simulink model "HPP"  (R2026a)
settings: Solver=ode1  StopTime=p.sim.Tstop  FixedStep=HPP_Tnet
model workspace (MAT data in the model file):
  HPP_Tnet = 0.001
  HPP_Ts = 0.001
  HPP_delays = 1
  HPP_f0 = 50
  HPP_network = 1
  HPP_simscape = 1
  buildInfo.N_wt = 2
  buildInfo.N_pv = 2
  buildInfo.N_bess = 1
  buildInfo.built = "25-Nov-2026 18:23:45"
undefined symbols (not defined in the file): p
libraries: ee_lib x57, nesl_utility x29, fl_lib x6
(part 1 of 5)
Description:
  | Hierarchical HPP model, generated by utilities/build/buildHPP.m. Do not edit by hand: rebuild instead.
settings Model: Creator=kjaer  LastModifiedBy=kjaer
settings DataIOCC: Decimation=p.sim.logDecimation
settings DebuggingCC: AlgebraicLoopMsg=error

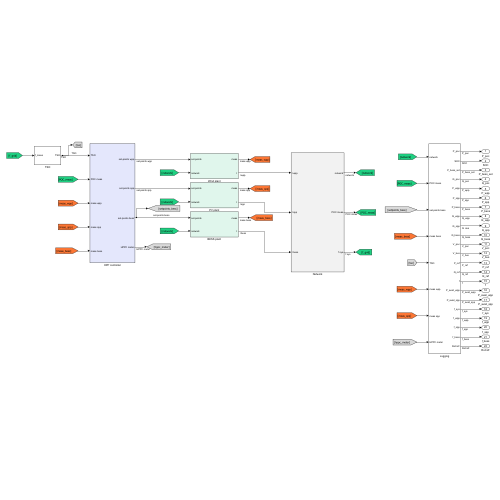
[thumbnail: Simulink's stored preview of the top-level diagram]
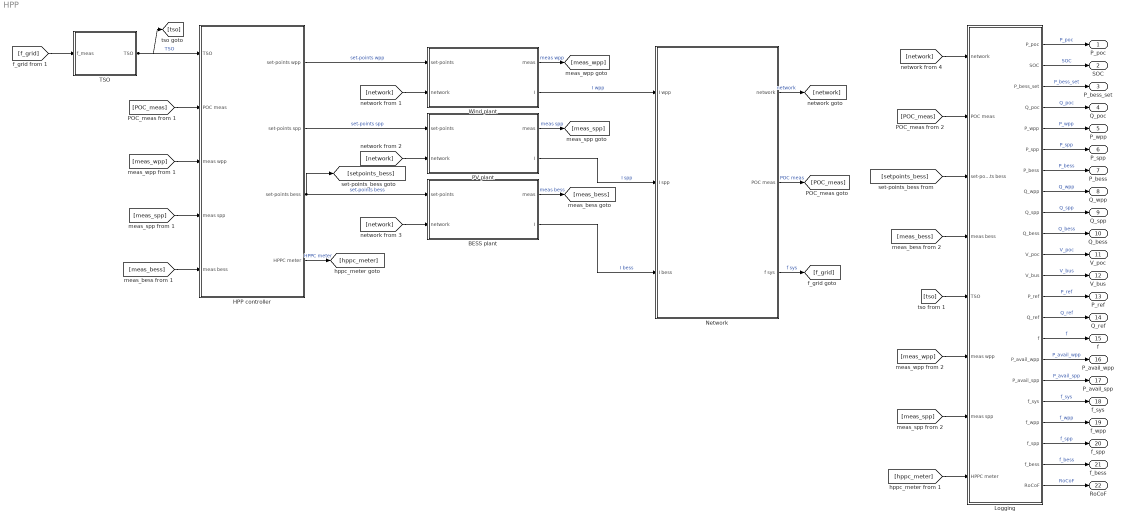
== system HPP ==
  BESS plant : Subsystem  Description=BESS plant: BESSC (plant controller) and 1 BESS asset instances. Bus interface in W / var; per-unit conversions and the delays of the links into this plant (p.comm) are inside. Local Goto/From: blue = set-points, green = network, orange = asset signals back to the plant controller.
  HPP controller : Subsystem  Description=HPP controller (HPPC.slx) with bus interface. Inputs in W / var / pu; converted to pu on p.ctrl.hppc.Pbase and delayed (p.comm) here. The HPPC's frequency meter (PLL on the POC voltage, p.pll.hppc) gives f_meas. Outputs: set-point buses in W / var; 4 meter bus (f, RoCoF) for logging.
  Logging : Subsystem  Description=Selects the logged signals (W, var, pu) for the top-level outports.
  Network : Subsystem  Description=Grid and network: Grid frequency (imposed or swing equation, angle of the grid source) and Network model (nodal or Simscape, chosen per run by HPP_network).
  PV plant : Subsystem  Description=PV plant: SPPC (plant controller) and 2 PV asset instances. Bus interface in W / var; per-unit conversions and the delays of the links into this plant (p.comm) are inside. Local Goto/From: blue = set-points, green = network, orange = asset signals back to the plant controller.
  TSO : Subsystem  Description=TSO / market set-points: P_ref [W], Q_ref [var]; f_meas [pu] passed on from the Grid frequency block.
  Wind plant : Subsystem  Description=Wind plant: WPPC (plant controller) and 2 WT asset instances. Bus interface in W / var; per-unit conversions and the delays of the links into this plant (p.comm) are inside. Local Goto/From: blue = set-points, green = network, orange = asset signals back to the plant controller.
  P_poc : Outport
  SOC : Outport  Port=2
  P_bess_set : Outport  Port=3
  Q_poc : Outport  Port=4
  P_wpp : Outport  Port=5
  P_spp : Outport  Port=6
  P_bess : Outport  Port=7
  Q_wpp : Outport  Port=8
  Q_spp : Outport  Port=9
  Q_bess : Outport  Port=10
  V_poc : Outport  Port=11
  V_bus : Outport  Port=12
  P_ref : Outport  Port=13
  Q_ref : Outport  Port=14
  f : Outport  Port=15
  P_avail_wpp : Outport  Port=16
  P_avail_spp : Outport  Port=17
  f_sys : Outport  Port=18
  f_wpp : Outport  Port=19
  f_spp : Outport  Port=20
  f_bess : Outport  Port=21
  RoCoF : Outport  Port=22
  wires:
  TSO/1(TSO) -> HPP controller/1(TSO), [tso]  "TSO"
  HPP controller/1(set-points wpp) -> Wind plant/1(set-points)  "set-points wpp"
  Wind plant/2(I) -> Network/1(I wpp)  "I wpp"
  HPP controller/2(set-points spp) -> PV plant/1(set-points)  "set-points spp"
  PV plant/2(I) -> Network/2(I spp)  "I spp"
  HPP controller/3(set-points bess) -> BESS plant/1(set-points), [setpoints_bess]  "set-points bess"
  BESS plant/2(I) -> Network/3(I bess)  "I bess"
  Wind plant/1(meas) -> [meas_wpp]  "meas wpp"
  [meas_wpp] -> HPP controller/3(meas wpp)
  [meas_wpp] -> Logging/6(meas wpp)
  PV plant/1(meas) -> [meas_spp]  "meas spp"
  [meas_spp] -> HPP controller/4(meas spp)
  [meas_spp] -> Logging/7(meas spp)
  [tso] -> Logging/5(TSO)
  BESS plant/1(meas) -> [meas_bess]  "meas bess"
  [meas_bess] -> HPP controller/5(meas bess)
  [meas_bess] -> Logging/4(meas bess)
  Network/1(network) -> [network]  "network"
  [network] -> Wind plant/2(network)
  [network] -> PV plant/2(network)
  [network] -> BESS plant/2(network)
  [network] -> Logging/1(network)
  Network/2(POC meas) -> [POC_meas]  "POC meas"
  [POC_meas] -> HPP controller/2(POC meas)
  [POC_meas] -> Logging/2(POC meas)
  Network/3(f sys) -> [f_grid]  "f sys"
  [f_grid] -> TSO/1(f_meas)
  HPP controller/4(HPPC meter) -> [hppc_meter]  "HPPC meter"
  [hppc_meter] -> Logging/8(HPPC meter)
  [setpoints_bess] -> Logging/3(set-points bess)
  Logging/1(P_poc) -> P_poc/1  "P_poc"
  Logging/2(SOC) -> SOC/1  "SOC"
  Logging/3(P_bess_set) -> P_bess_set/1  "P_bess_set"
  Logging/4(Q_poc) -> Q_poc/1  "Q_poc"
  Logging/5(P_wpp) -> P_wpp/1  "P_wpp"
  Logging/6(P_spp) -> P_spp/1  "P_spp"
  Logging/7(P_bess) -> P_bess/1  "P_bess"
  Logging/8(Q_wpp) -> Q_wpp/1  "Q_wpp"
  Logging/9(Q_spp) -> Q_spp/1  "Q_spp"
  Logging/10(Q_bess) -> Q_bess/1  "Q_bess"
  Logging/11(V_poc) -> V_poc/1  "V_poc"
  Logging/12(V_bus) -> V_bus/1  "V_bus"
  Logging/13(P_ref) -> P_ref/1  "P_ref"
  Logging/14(Q_ref) -> Q_ref/1  "Q_ref"
  Logging/15(f) -> f/1  "f"
  Logging/16(P_avail_wpp) -> P_avail_wpp/1  "P_avail_wpp"
  Logging/17(P_avail_spp) -> P_avail_spp/1  "P_avail_spp"
  Logging/18(f_sys) -> f_sys/1  "f_sys"
  Logging/19(f_wpp) -> f_wpp/1  "f_wpp"
  Logging/20(f_spp) -> f_spp/1  "f_spp"
  Logging/21(f_bess) -> f_bess/1  "f_bess"
  Logging/22(RoCoF) -> RoCoF/1  "RoCoF"

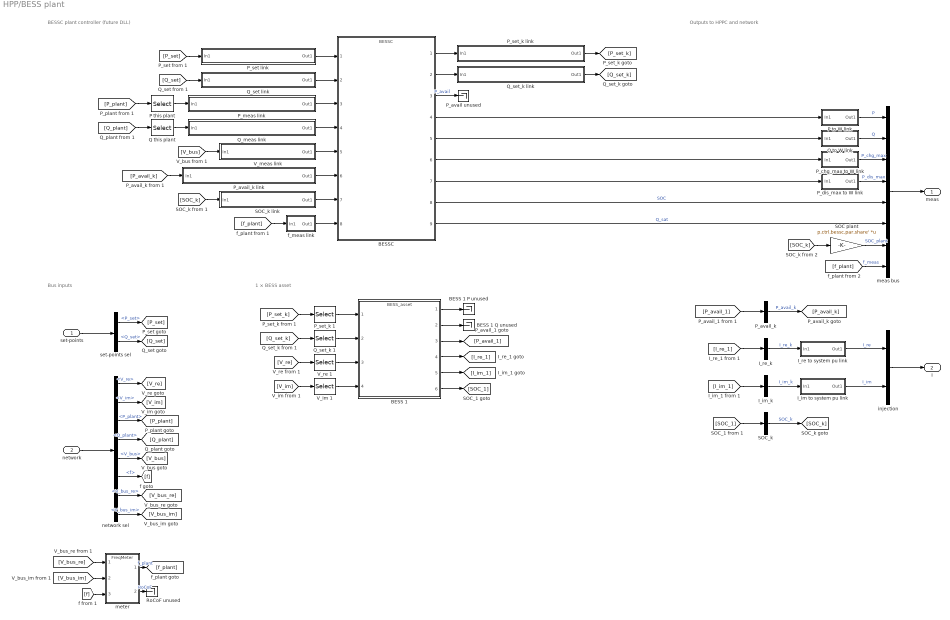
== system HPP/BESS plant ==
  note: Bus inputs
  note: BESSC plant controller (future DLL)
  note: 1 × BESS asset
  note: Outputs to HPPC and network
  set-points : Inport
  network : Inport  Port=2
  BESS 1 : ModelReference  ModelNameDialog=BESS_asset  ParameterArgumentNames=ap  ParameterArgumentValues=p.bess.ap(1)  UsingDefaultArgumentValue=0  SimulationMode=Normal  ModelReferenceVersion=1.1
  BESS 1 P unused : Terminator
  BESS 1 Q unused : Terminator
  BESSC : ModelReference  ModelNameDialog=BESSC  ParameterArgumentNames=par  ParameterArgumentValues=p.ctrl.bessc.par  UsingDefaultArgumentValue=0  SimulationMode=Normal  ModelReferenceVersion=1.1
  I_im to system pu link : Subsystem
      mask help: Link: gain p.ctrl.bess.Pbase/p.grid.Pbase.
      mask Display: disp('pu base')
  I_im_k : Mux  Inputs=1
  I_re to system pu link : Subsystem
      mask help: Link: gain p.ctrl.bess.Pbase/p.grid.Pbase.
      mask Display: disp('pu base')
  I_re_k : Mux  Inputs=1
  P this plant : Selector  InputPortWidth=3  IndexOptions=Index vector (dialog)  Indices=3  OutputSizes=1
  P to W link : Subsystem
      mask help: Link: gain p.ctrl.bessc.Pbase.
      mask Display: disp('to SI')
  P_avail unused : Terminator
  P_avail_k : Mux  Inputs=1
  P_avail_k link : Subsystem
      mask help: Link: gain p.ctrl.bess.Pbase/p.ctrl.bessc.Pbase, then one-step memory, then delay p.comm.meas_plant in whole steps (initial output 0).
      mask Display: disp('pu base | mem | comm.meas_plant')
  P_chg_max to W link : Subsystem
      mask help: Link: gain p.ctrl.bessc.Pbase.
      mask Display: disp('to SI')
  P_dis_max to W link : Subsystem
      mask help: Link: gain p.ctrl.bessc.Pbase.
      mask Display: disp('to SI')
  P_meas link : Subsystem
      mask help: Link: gain 1/p.ctrl.bessc.Pbase, then one-step memory, then delay p.comm.meas_plant in whole steps (initial output 0).
      mask Display: disp('to pu | mem | comm.meas_plant')
  P_set link : Subsystem
      mask help: Link: delay p.comm.hppc_to_plant in whole steps (initial output 0), then gain 1/p.ctrl.bessc.Pbase.
      mask Display: disp('comm.hppc_to_plant | to pu')
  P_set_k 1 : Selector  InputPortWidth=1  IndexOptions=Index vector (dialog)  Indices=1  OutputSizes=1
  P_set_k link : Subsystem
      mask help: Link: delay p.comm.plant_to_asset in whole steps (initial output 0), then gain p.ctrl.bessc.Pbase/p.ctrl.bess.Pbase.
      mask Display: disp('comm.plant_to_asset | pu base')
  Q this plant : Selector  InputPortWidth=3  IndexOptions=Index vector (dialog)  Indices=3  OutputSizes=1
  Q to W link : Subsystem
      mask help: Link: gain p.ctrl.bessc.Pbase.
      mask Display: disp('to SI')
  Q_meas link : Subsystem
      mask help: Link: gain 1/p.ctrl.bessc.Pbase, then one-step memory, then delay p.comm.meas_plant in whole steps (initial output 0).
      mask Display: disp('to pu | mem | comm.meas_plant')
  Q_set link : Subsystem
      mask help: Link: delay p.comm.hppc_to_plant in whole steps (initial output 0), then gain 1/p.ctrl.bessc.Pbase.
      mask Display: disp('comm.hppc_to_plant | to pu')
  Q_set_k 1 : Selector  InputPortWidth=1  IndexOptions=Index vector (dialog)  Indices=1  OutputSizes=1
  Q_set_k link : Subsystem
      mask help: Link: delay p.comm.plant_to_asset in whole steps (initial output 0), then gain p.ctrl.bessc.Pbase/p.ctrl.bess.Pbase.
      mask Display: disp('comm.plant_to_asset | pu base')
  RoCoF unused : Terminator
  SOC plant : Gain  Gain=p.ctrl.bessc.par.share'  Multiplication=Matrix(K*u)
  SOC_k : Mux  Inputs=1
  SOC_k link : Subsystem
      mask help: Link: one-step memory, then delay p.comm.meas_plant in whole steps (initial output 0).
      mask Display: disp('mem | comm.meas_plant')
  V_im 1 : Selector  InputPortWidth=5  IndexOptions=Index vector (dialog)  Indices=5  OutputSizes=1
  V_meas link : Subsystem
      mask help: Link: one-step memory, then delay p.comm.meas_plant in whole steps (initial output 1).
      mask Display: disp('mem | comm.meas_plant')
  V_re 1 : Selector  InputPortWidth=5  IndexOptions=Index vector (dialog)  Indices=5  OutputSizes=1
  f_meas link : Subsystem
      mask help: Link: one-step memory.
      mask Display: disp('mem')
  injection : BusCreator  Inputs=2
  meas bus : BusCreator  Inputs=8
  meter : ModelReference  ModelNameDialog=FreqMeter  ParameterArgumentNames=m  ParameterArgumentValues=p.pll.bessc  UsingDefaultArgumentValue=0  SimulationMode=Normal  ModelReferenceVersion=1.1
  network sel : BusSelector  OutputSignals=V_re,V_im,P_plant,Q_plant,V_bus,f,V_bus_re,V_bus_im
  set-points sel : BusSelector  OutputSignals=P_set,Q_set
  meas : Outport
  I : Outport  Port=2
  wires:
  set-points/1 -> set-points sel/1
  network/1 -> network sel/1
  set-points sel/1 -> [P_set]  "<P_set>"
  set-points sel/2 -> [Q_set]  "<Q_set>"
  network sel/1 -> [V_re]  "<V_re>"
  network sel/2 -> [V_im]  "<V_im>"
  network sel/3 -> [P_plant]  "<P_plant>"
  network sel/4 -> [Q_plant]  "<Q_plant>"
  network sel/5 -> [V_bus]  "<V_bus>"
  network sel/6 -> [f]  "<f>"
  network sel/7 -> [V_bus_re]  "<V_bus_re>"
  network sel/8 -> [V_bus_im]  "<V_bus_im>"
  [P_set] -> P_set link/1(In1)
  P_set link/1(Out1) -> BESSC/1
  [Q_set] -> Q_set link/1(In1)
  Q_set link/1(Out1) -> BESSC/2
  [P_plant] -> P this plant/1
  P this plant/1 -> P_meas link/1(In1)
  P_meas link/1(Out1) -> BESSC/3
  [Q_plant] -> Q this plant/1
  Q this plant/1 -> Q_meas link/1(In1)
  Q_meas link/1(Out1) -> BESSC/4
  [V_bus] -> V_meas link/1(In1)
  V_meas link/1(Out1) -> BESSC/5
  [P_avail_k] -> P_avail_k link/1(In1)
  P_avail_k link/1(Out1) -> BESSC/6
  [SOC_k] -> SOC_k link/1(In1)
  SOC_k link/1(Out1) -> BESSC/7
  [V_bus_re] -> meter/1
  [V_bus_im] -> meter/2
  [f] -> meter/3
  meter/1 -> [f_plant]  "f_plant"
  meter/2 -> RoCoF unused/1  "RoCoF"
  [f_plant] -> f_meas link/1(In1)
  f_meas link/1(Out1) -> BESSC/8
  BESSC/1 -> P_set_k link/1(In1)
  P_set_k link/1(Out1) -> [P_set_k]
  BESSC/2 -> Q_set_k link/1(In1)
  Q_set_k link/1(Out1) -> [Q_set_k]
  [P_set_k] -> P_set_k 1/1
  P_set_k 1/1 -> BESS 1/1
  [Q_set_k] -> Q_set_k 1/1
  Q_set_k 1/1 -> BESS 1/2
  [V_re] -> V_re 1/1
  V_re 1/1 -> BESS 1/3
  [V_im] -> V_im 1/1
  V_im 1/1 -> BESS 1/4
  BESS 1/1 -> BESS 1 P unused/1
  BESS 1/2 -> BESS 1 Q unused/1
  BESS 1/3 -> [P_avail_1]
  BESS 1/4 -> [I_re_1]
  BESS 1/5 -> [I_im_1]
  BESS 1/6 -> [SOC_1]
  [P_avail_1] -> P_avail_k/1
  [I_re_1] -> I_re_k/1
  [I_im_1] -> I_im_k/1
  [SOC_1] -> SOC_k/1
  P_avail_k/1 -> [P_avail_k]  "P_avail_k"
  I_re_k/1 -> I_re to system pu link/1(In1)  "I_re_k"
  I_im_k/1 -> I_im to system pu link/1(In1)  "I_im_k"
  I_re to system pu link/1(Out1) -> injection/1  "I_re"
  I_im to system pu link/1(Out1) -> injection/2  "I_im"
  injection/1 -> I/1
  SOC_k/1 -> [SOC_k]  "SOC_k"
  BESSC/3 -> P_avail unused/1  "P_avail"
  BESSC/4 -> P to W link/1(In1)
  P to W link/1(Out1) -> meas bus/1  "P"
  BESSC/5 -> Q to W link/1(In1)
  Q to W link/1(Out1) -> meas bus/2  "Q"
  BESSC/6 -> P_chg_max to W link/1(In1)
  P_chg_max to W link/1(Out1) -> meas bus/3  "P_chg_max"
  BESSC/7 -> P_dis_max to W link/1(In1)
  P_dis_max to W link/1(Out1) -> meas bus/4  "P_dis_max"
  BESSC/8 -> meas bus/5  "SOC"
  BESSC/9 -> meas bus/6  "Q_sat"
  [SOC_k] -> SOC plant/1
  SOC plant/1 -> meas bus/7  "SOC_plant"
  [f_plant] -> meas bus/8  "f_meas"
  meas bus/1 -> meas/1

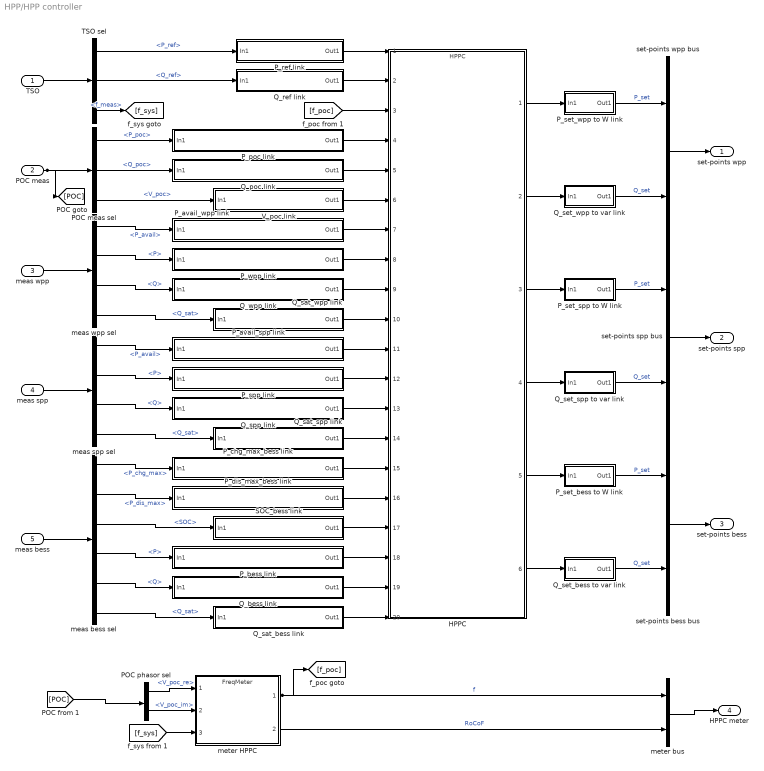
== system HPP/HPP controller ==
  TSO : Inport
  POC meas : Inport  Port=2
  meas wpp : Inport  Port=3
  meas spp : Inport  Port=4
  meas bess : Inport  Port=5
  HPPC : ModelReference  ModelNameDialog=HPPC  ParameterArgumentNames=par  ParameterArgumentValues=p.ctrl.hppc.par  UsingDefaultArgumentValue=0  SimulationMode=Normal  ModelReferenceVersion=1.1
  POC meas sel : BusSelector  OutputSignals=P_poc,Q_poc,V_poc
  POC phasor sel : BusSelector  OutputSignals=V_poc_re,V_poc_im
  P_avail_spp link : Subsystem
      mask help: Link: gain 1/p.ctrl.hppc.Pbase, then one-step memory, then delay p.comm.meas_hppc in whole steps (initial output 0).
      mask Display: disp('to pu | mem | comm.meas_hppc')
  P_avail_wpp link : Subsystem
      mask help: Link: gain 1/p.ctrl.hppc.Pbase, then one-step memory, then delay p.comm.meas_hppc in whole steps (initial output 0).
      mask Display: disp('to pu | mem | comm.meas_hppc')
  P_bess link : Subsystem
      mask help: Link: gain 1/p.ctrl.hppc.Pbase, then one-step memory, then delay p.comm.meas_hppc in whole steps (initial output 0).
      mask Display: disp('to pu | mem | comm.meas_hppc')
  P_chg_max_bess link : Subsystem
      mask help: Link: gain 1/p.ctrl.hppc.Pbase, then one-step memory, then delay p.comm.meas_hppc in whole steps (initial output 0).
      mask Display: disp('to pu | mem | comm.meas_hppc')
  P_dis_max_bess link : Subsystem
      mask help: Link: gain 1/p.ctrl.hppc.Pbase, then one-step memory, then delay p.comm.meas_hppc in whole steps (initial output 0).
      mask Display: disp('to pu | mem | comm.meas_hppc')
  P_poc link : Subsystem
      mask help: Link: gain 1/p.ctrl.hppc.Pbase, then one-step memory, then delay p.comm.meas_hppc in whole steps (initial output 0).
      mask Display: disp('to pu | mem | comm.meas_hppc')
  P_ref link : Subsystem
      mask help: Link: gain 1/p.ctrl.hppc.Pbase, then delay p.comm.tso in whole steps (initial output p.grid.Pref/p.ctrl.hppc.Pbase).
      mask Display: disp('to pu | comm.tso')
  P_set_bess to W link : Subsystem
      mask help: Link: gain p.ctrl.hppc.Pbase.
      mask Display: disp('to SI')
  P_set_spp to W link : Subsystem
      mask help: Link: gain p.ctrl.hppc.Pbase.
      mask Display: disp('to SI')
  P_set_wpp to W link : Subsystem
      mask help: Link: gain p.ctrl.hppc.Pbase.
      mask Display: disp('to SI')
  P_spp link : Subsystem
      mask help: Link: gain 1/p.ctrl.hppc.Pbase, then one-step memory, then delay p.comm.meas_hppc in whole steps (initial output 0).
      mask Display: disp('to pu | mem | comm.meas_hppc')
  P_wpp link : Subsystem
      mask help: Link: gain 1/p.ctrl.hppc.Pbase, then one-step memory, then delay p.comm.meas_hppc in whole steps (initial output 0).
      mask Display: disp('to pu | mem | comm.meas_hppc')
  Q_bess link : Subsystem
      mask help: Link: gain 1/p.ctrl.hppc.Pbase, then one-step memory, then delay p.comm.meas_hppc in whole steps (initial output 0).
      mask Display: disp('to pu | mem | comm.meas_hppc')
  Q_poc link : Subsystem
      mask help: Link: gain 1/p.ctrl.hppc.Pbase, then one-step memory, then delay p.comm.meas_hppc in whole steps (initial output 0).
      mask Display: disp('to pu | mem | comm.meas_hppc')
  Q_ref link : Subsystem
      mask help: Link: gain 1/p.ctrl.hppc.Pbase, then delay p.comm.tso in whole steps (initial output p.grid.Qref/p.ctrl.hppc.Pbase).
      mask Display: disp('to pu | comm.tso')
  Q_sat_bess link : Subsystem
      mask help: Link: one-step memory, then delay p.comm.meas_hppc in whole steps (initial output 0).
      mask Display: disp('mem | comm.meas_hppc')
  Q_sat_spp link : Subsystem
      mask help: Link: one-step memory, then delay p.comm.meas_hppc in whole steps (initial output 0).
      mask Display: disp('mem | comm.meas_hppc')
  Q_sat_wpp link : Subsystem
      mask help: Link: one-step memory, then delay p.comm.meas_hppc in whole steps (initial output 0).
      mask Display: disp('mem | comm.meas_hppc')
  Q_set_bess to var link : Subsystem
      mask help: Link: gain p.ctrl.hppc.Pbase.
      mask Display: disp('to SI')
  Q_set_spp to var link : Subsystem
      mask help: Link: gain p.ctrl.hppc.Pbase.
      mask Display: disp('to SI')
  Q_set_wpp to var link : Subsystem
      mask help: Link: gain p.ctrl.hppc.Pbase.
      mask Display: disp('to SI')
  Q_spp link : Subsystem
      mask help: Link: gain 1/p.ctrl.hppc.Pbase, then one-step memory, then delay p.comm.meas_hppc in whole steps (initial output 0).
      mask Display: disp('to pu | mem | comm.meas_hppc')
  Q_wpp link : Subsystem
      mask help: Link: gain 1/p.ctrl.hppc.Pbase, then one-step memory, then delay p.comm.meas_hppc in whole steps (initial output 0).
      mask Display: disp('to pu | mem | comm.meas_hppc')
  SOC_bess link : Subsystem
      mask help: Link: one-step memory, then delay p.comm.meas_hppc in whole steps (initial output 0).
      mask Display: disp('mem | comm.meas_hppc')
  TSO sel : BusSelector  OutputSignals=P_ref,Q_ref,f_meas
  V_poc link : Subsystem
      mask help: Link: one-step memory, then delay p.comm.meas_hppc in whole steps (initial output 1).
      mask Display: disp('mem | comm.meas_hppc')
  meas bess sel : BusSelector  OutputSignals=P_chg_max,P_dis_max,SOC,P,Q,Q_sat
  meas spp sel : BusSelector  OutputSignals=P_avail,P,Q,Q_sat
  meas wpp sel : BusSelector  OutputSignals=P_avail,P,Q,Q_sat
  meter HPPC : ModelReference  ModelNameDialog=FreqMeter  ParameterArgumentNames=m  ParameterArgumentValues=p.pll.hppc  UsingDefaultArgumentValue=0  SimulationMode=Normal  ModelReferenceVersion=1.1
  meter bus : BusCreator  Inputs=2
  set-points bess bus : BusCreator  Inputs=2
  set-points spp bus : BusCreator  Inputs=2
  set-points wpp bus : BusCreator  Inputs=2
  set-points wpp : Outport
  set-points spp : Outport  Port=2
  set-points bess : Outport  Port=3
  HPPC meter : Outport  Port=4
  wires:
  TSO/1 -> TSO sel/1
  P_ref link/1(Out1) -> HPPC/1
  TSO sel/1 -> P_ref link/1(In1)  "<P_ref>"
  Q_ref link/1(Out1) -> HPPC/2
  TSO sel/2 -> Q_ref link/1(In1)  "<Q_ref>"
  TSO sel/3 -> [f_sys]  "<f_meas>"
  [f_poc] -> HPPC/3
  POC meas/1 -> POC meas sel/1, [POC]
  P_poc link/1(Out1) -> HPPC/4
  POC meas sel/1 -> P_poc link/1(In1)  "<P_poc>"
  Q_poc link/1(Out1) -> HPPC/5
  POC meas sel/2 -> Q_poc link/1(In1)  "<Q_poc>"
  V_poc link/1(Out1) -> HPPC/6
  POC meas sel/3 -> V_poc link/1(In1)  "<V_poc>"
  meas wpp/1 -> meas wpp sel/1
  P_avail_wpp link/1(Out1) -> HPPC/7
  meas wpp sel/1 -> P_avail_wpp link/1(In1)  "<P_avail>"
  P_wpp link/1(Out1) -> HPPC/8
  meas wpp sel/2 -> P_wpp link/1(In1)  "<P>"
  Q_wpp link/1(Out1) -> HPPC/9
  meas wpp sel/3 -> Q_wpp link/1(In1)  "<Q>"
  Q_sat_wpp link/1(Out1) -> HPPC/10
  meas wpp sel/4 -> Q_sat_wpp link/1(In1)  "<Q_sat>"
  meas spp/1 -> meas spp sel/1
  P_avail_spp link/1(Out1) -> HPPC/11
  meas spp sel/1 -> P_avail_spp link/1(In1)  "<P_avail>"
  P_spp link/1(Out1) -> HPPC/12
  meas spp sel/2 -> P_spp link/1(In1)  "<P>"
  Q_spp link/1(Out1) -> HPPC/13
  meas spp sel/3 -> Q_spp link/1(In1)  "<Q>"
  Q_sat_spp link/1(Out1) -> HPPC/14
  meas spp sel/4 -> Q_sat_spp link/1(In1)  "<Q_sat>"
  meas bess/1 -> meas bess sel/1
  P_chg_max_bess link/1(Out1) -> HPPC/15
  meas bess sel/1 -> P_chg_max_bess link/1(In1)  "<P_chg_max>"
  P_dis_max_bess link/1(Out1) -> HPPC/16
  meas bess sel/2 -> P_dis_max_bess link/1(In1)  "<P_dis_max>"
  SOC_bess link/1(Out1) -> HPPC/17
  meas bess sel/3 -> SOC_bess link/1(In1)  "<SOC>"
  P_bess link/1(Out1) -> HPPC/18
  meas bess sel/4 -> P_bess link/1(In1)  "<P>"
  Q_bess link/1(Out1) -> HPPC/19
  meas bess sel/5 -> Q_bess link/1(In1)  "<Q>"
  Q_sat_bess link/1(Out1) -> HPPC/20
  meas bess sel/6 -> Q_sat_bess link/1(In1)  "<Q_sat>"
  HPPC/1 -> P_set_wpp to W link/1(In1)
  P_set_wpp to W link/1(Out1) -> set-points wpp bus/1  "P_set"
  HPPC/2 -> Q_set_wpp to var link/1(In1)
  Q_set_wpp to var link/1(Out1) -> set-points wpp bus/2  "Q_set"
  set-points wpp bus/1 -> set-points wpp/1
  HPPC/3 -> P_set_spp to W link/1(In1)
  P_set_spp to W link/1(Out1) -> set-points spp bus/1  "P_set"
  HPPC/4 -> Q_set_spp to var link/1(In1)
  Q_set_spp to var link/1(Out1) -> set-points spp bus/2  "Q_set"
  set-points spp bus/1 -> set-points spp/1
  HPPC/5 -> P_set_bess to W link/1(In1)
  P_set_bess to W link/1(Out1) -> set-points bess bus/1  "P_set"
  HPPC/6 -> Q_set_bess to var link/1(In1)
  Q_set_bess to var link/1(Out1) -> set-points bess bus/2  "Q_set"
  set-points bess bus/1 -> set-points bess/1
  [POC] -> POC phasor sel/1
  POC phasor sel/1 -> meter HPPC/1  "<V_poc_re>"
  POC phasor sel/2 -> meter HPPC/2  "<V_poc_im>"
  [f_sys] -> meter HPPC/3
  meter HPPC/1 -> [f_poc], meter bus/1  "f"
  meter HPPC/2 -> meter bus/2  "RoCoF"
  meter bus/1 -> HPPC meter/1

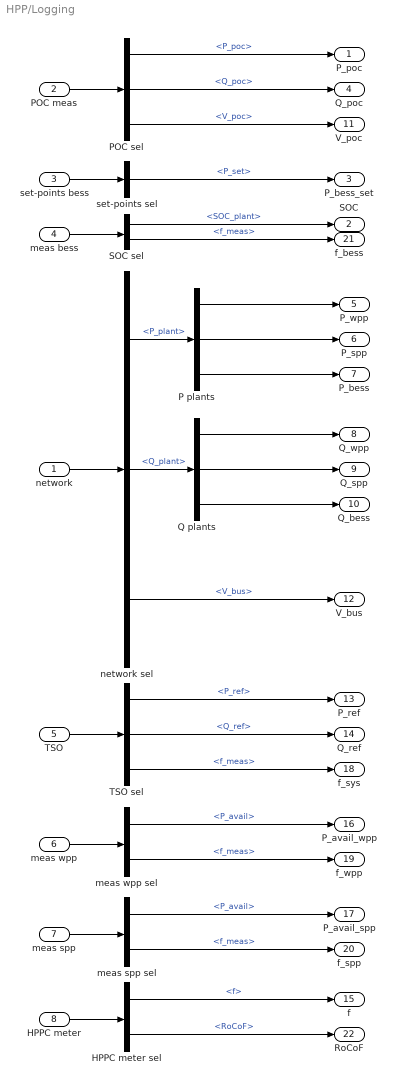
== system HPP/Logging ==
  network : Inport
  POC meas : Inport  Port=2
  set-points bess : Inport  Port=3
  meas bess : Inport  Port=4
  TSO : Inport  Port=5
  meas wpp : Inport  Port=6
  meas spp : Inport  Port=7
  HPPC meter : Inport  Port=8
  HPPC meter sel : BusSelector  OutputSignals=f,RoCoF
  P plants : Demux  Outputs=3
  POC sel : BusSelector  OutputSignals=P_poc,Q_poc,V_poc
  Q plants : Demux  Outputs=3
  SOC sel : BusSelector  OutputSignals=SOC_plant,f_meas
  TSO sel : BusSelector  OutputSignals=P_ref,Q_ref,f_meas
  meas spp sel : BusSelector  OutputSignals=P_avail,f_meas
  meas wpp sel : BusSelector  OutputSignals=P_avail,f_meas
  network sel : BusSelector  OutputSignals=P_plant,Q_plant,V_bus
  set-points sel : BusSelector  OutputSignals=P_set
  P_poc : Outport
  SOC : Outport  Port=2
  P_bess_set : Outport  Port=3
  Q_poc : Outport  Port=4
  P_wpp : Outport  Port=5
  P_spp : Outport  Port=6
  P_bess : Outport  Port=7
  Q_wpp : Outport  Port=8
  Q_spp : Outport  Port=9
  Q_bess : Outport  Port=10
  V_poc : Outport  Port=11
  V_bus : Outport  Port=12
  P_ref : Outport  Port=13
  Q_ref : Outport  Port=14
  f : Outport  Port=15
  P_avail_wpp : Outport  Port=16
  P_avail_spp : Outport  Port=17
  f_sys : Outport  Port=18
  f_wpp : Outport  Port=19
  f_spp : Outport  Port=20
  f_bess : Outport  Port=21
  RoCoF : Outport  Port=22
  wires:
  POC meas/1 -> POC sel/1
  POC sel/1 -> P_poc/1  "<P_poc>"
  POC sel/2 -> Q_poc/1  "<Q_poc>"
  POC sel/3 -> V_poc/1  "<V_poc>"
  set-points bess/1 -> set-points sel/1
  set-points sel/1 -> P_bess_set/1  "<P_set>"
  meas bess/1 -> SOC sel/1
  SOC sel/1 -> SOC/1  "<SOC_plant>"
  SOC sel/2 -> f_bess/1  "<f_meas>"
  network/1 -> network sel/1
  network sel/1 -> P plants/1  "<P_plant>"
  P plants/1 -> P_wpp/1
  P plants/2 -> P_spp/1
  P plants/3 -> P_bess/1
  network sel/2 -> Q plants/1  "<Q_plant>"
  Q plants/1 -> Q_wpp/1
  Q plants/2 -> Q_spp/1
  Q plants/3 -> Q_bess/1
  network sel/3 -> V_bus/1  "<V_bus>"
  TSO/1 -> TSO sel/1
  TSO sel/1 -> P_ref/1  "<P_ref>"
  TSO sel/2 -> Q_ref/1  "<Q_ref>"
  TSO sel/3 -> f_sys/1  "<f_meas>"
  meas wpp/1 -> meas wpp sel/1
  meas wpp sel/1 -> P_avail_wpp/1  "<P_avail>"
  meas wpp sel/2 -> f_wpp/1  "<f_meas>"
  meas spp/1 -> meas spp sel/1
  meas spp sel/1 -> P_avail_spp/1  "<P_avail>"
  meas spp sel/2 -> f_spp/1  "<f_meas>"
  HPPC meter/1 -> HPPC meter sel/1
  HPPC meter sel/1 -> f/1  "<f>"
  HPPC meter sel/2 -> RoCoF/1  "<RoCoF>"

== system HPP/Network ==
  I wpp : Inport
  I spp : Inport  Port=2
  I bess : Inport  Port=3
  Grid frequency : Subsystem  TreatAsAtomicUnit=on  SystemSampleTime=p.sim.Ts  mask{g=p.grid}
      mask prompts: g "Grid data"
      mask help: Grid frequency [pu] and angle [rad]: imposed (p.grid.fev, p.grid.fprof) or swing equation (p.grid.sys.swing = 1). See params/gridParameters.m.
      mask Display: disp('grid frequency')
  Network model : Subsystem  Description=Network model, chosen per run: Nodal (HPP_network = 1, fast nodal solver) or Simscape (HPP_network = 2, Simscape Electrical, phasor or EMT mode by HPP_simscape). See runCase, option Network.  Variant=on
  network : Outport
  POC meas : Outport  Port=2
  f sys : Outport  Port=3
  wires:
  I wpp/1 -> Network model/1(I wpp)  "I wpp"
  I spp/1 -> Network model/2(I spp)  "I spp"
  I bess/1 -> Network model/3(I bess)  "I bess"
  Grid frequency/1(f) -> Network model/4(f grid), [f_sys]  "f"
  Grid frequency/2(theta) -> Network model/5(theta)  "theta"
  Network model/1(network) -> network/1  "network"
  Network model/2(POC meas) -> POC meas/1, [POC_fb]  "POC meas"
  [POC_fb] -> Grid frequency/1(POC meas)
  [f_sys] -> f sys/1

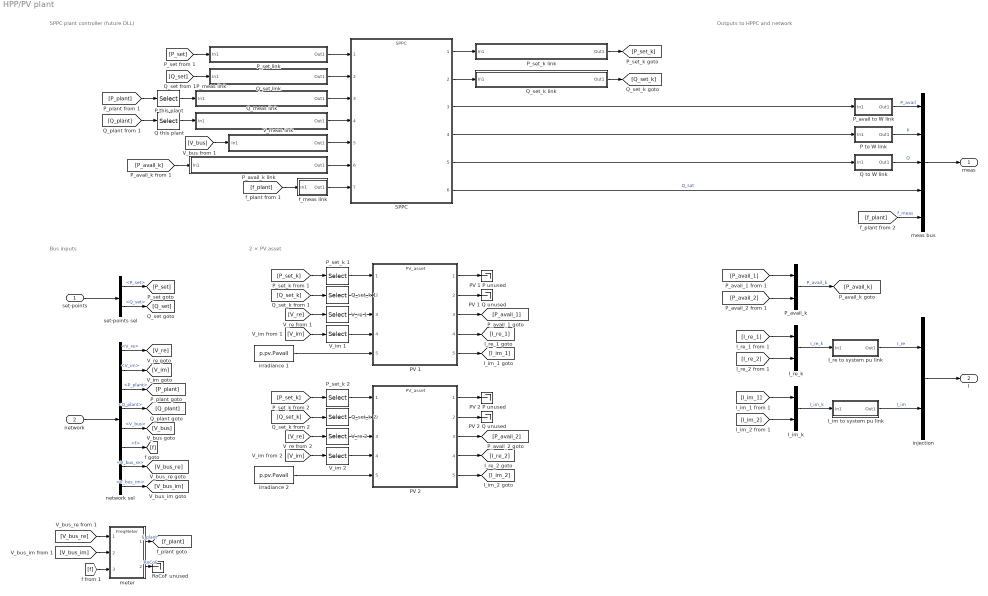
== system HPP/PV plant ==
  note: Bus inputs
  note: SPPC plant controller (future DLL)
  note: 2 × PV asset
  note: Outputs to HPPC and network
  set-points : Inport
  network : Inport  Port=2
  I_im to system pu link : Subsystem
      mask help: Link: gain p.ctrl.pv.Pbase/p.grid.Pbase.
      mask Display: disp('pu base')
  I_im_k : Mux  Inputs=2
  I_re to system pu link : Subsystem
      mask help: Link: gain p.ctrl.pv.Pbase/p.grid.Pbase.
      mask Display: disp('pu base')
  I_re_k : Mux  Inputs=2
  P this plant : Selector  InputPortWidth=3  IndexOptions=Index vector (dialog)  Indices=2  OutputSizes=1
  P to W link : Subsystem
      mask help: Link: gain p.ctrl.sppc.Pbase.
      mask Display: disp('to SI')
  PV 1 : ModelReference  ModelNameDialog=PV_asset  ParameterArgumentNames=ap  ParameterArgumentValues=p.pv.ap(1)  UsingDefaultArgumentValue=0  SimulationMode=Normal  ModelReferenceVersion=1.1
  PV 1 P unused : Terminator
  PV 1 Q unused : Terminator
  PV 2 : ModelReference  ModelNameDialog=PV_asset  ParameterArgumentNames=ap  ParameterArgumentValues=p.pv.ap(2)  UsingDefaultArgumentValue=0  SimulationMode=Normal  ModelReferenceVersion=1.1
  PV 2 P unused : Terminator
  PV 2 Q unused : Terminator
  P_avail to W link : Subsystem
      mask help: Link: gain p.ctrl.sppc.Pbase.
      mask Display: disp('to SI')
  P_avail_k : Mux  Inputs=2
  P_avail_k link : Subsystem
      mask help: Link: gain p.ctrl.pv.Pbase/p.ctrl.sppc.Pbase, then one-step memory, then delay p.comm.meas_plant in whole steps (initial output 0).
      mask Display: disp('pu base | mem | comm.meas_plant')
  P_meas link : Subsystem
      mask help: Link: gain 1/p.ctrl.sppc.Pbase, then one-step memory, then delay p.comm.meas_plant in whole steps (initial output 0).
      mask Display: disp('to pu | mem | comm.meas_plant')
  P_set link : Subsystem
      mask help: Link: delay p.comm.hppc_to_plant in whole steps (initial output 0), then gain 1/p.ctrl.sppc.Pbase.
      mask Display: disp('comm.hppc_to_plant | to pu')
  P_set_k 1 : Selector  InputPortWidth=2  IndexOptions=Index vector (dialog)  Indices=1  OutputSizes=1
  P_set_k 2 : Selector  InputPortWidth=2  IndexOptions=Index vector (dialog)  Indices=2  OutputSizes=1
  P_set_k link : Subsystem
      mask help: Link: delay p.comm.plant_to_asset in whole steps (initial output 0), then gain p.ctrl.sppc.Pbase/p.ctrl.pv.Pbase.
      mask Display: disp('comm.plant_to_asset | pu base')
  Q this plant : Selector  InputPortWidth=3  IndexOptions=Index vector (dialog)  Indices=2  OutputSizes=1
  Q to W link : Subsystem
      mask help: Link: gain p.ctrl.sppc.Pbase.
      mask Display: disp('to SI')
  Q_meas link : Subsystem
      mask help: Link: gain 1/p.ctrl.sppc.Pbase, then one-step memory, then delay p.comm.meas_plant in whole steps (initial output 0).
      mask Display: disp('to pu | mem | comm.meas_plant')
  Q_set link : Subsystem
      mask help: Link: delay p.comm.hppc_to_plant in whole steps (initial output 0), then gain 1/p.ctrl.sppc.Pbase.
      mask Display: disp('comm.hppc_to_plant | to pu')
  Q_set_k 1 : Selector  InputPortWidth=2  IndexOptions=Index vector (dialog)  Indices=1  OutputSizes=1
  Q_set_k 2 : Selector  InputPortWidth=2  IndexOptions=Index vector (dialog)  Indices=2  OutputSizes=1
  Q_set_k link : Subsystem
      mask help: Link: delay p.comm.plant_to_asset in whole steps (initial output 0), then gain p.ctrl.sppc.Pbase/p.ctrl.pv.Pbase.
      mask Display: disp('comm.plant_to_asset | pu base')
  RoCoF unused : Terminator
  SPPC : ModelReference  ModelNameDialog=SPPC  ParameterArgumentNames=par  ParameterArgumentValues=p.ctrl.sppc.par  UsingDefaultArgumentValue=0  SimulationMode=Normal  ModelReferenceVersion=1.1
  V_im 1 : Selector  InputPortWidth=5  IndexOptions=Index vector (dialog)  Indices=3  OutputSizes=1
  V_im 2 : Selector  InputPortWidth=5  IndexOptions=Index vector (dialog)  Indices=4  OutputSizes=1
  V_meas link : Subsystem
      mask help: Link: one-step memory, then delay p.comm.meas_plant in whole steps (initial output 1).
      mask Display: disp('mem | comm.meas_plant')
  V_re 1 : Selector  InputPortWidth=5  IndexOptions=Index vector (dialog)  Indices=3  OutputSizes=1
  V_re 2 : Selector  InputPortWidth=5  IndexOptions=Index vector (dialog)  Indices=4  OutputSizes=1
  f_meas link : Subsystem
      mask help: Link: one-step memory.
      mask Display: disp('mem')
  injection : BusCreator  Inputs=2
  irradiance 1 : Constant  Value=p.pv.Pavail
  irradiance 2 : Constant  Value=p.pv.Pavail
  meas bus : BusCreator  Inputs=5
  meter : ModelReference  ModelNameDialog=FreqMeter  ParameterArgumentNames=m  ParameterArgumentValues=p.pll.sppc  UsingDefaultArgumentValue=0  SimulationMode=Normal  ModelReferenceVersion=1.1
  network sel : BusSelector  OutputSignals=V_re,V_im,P_plant,Q_plant,V_bus,f,V_bus_re,V_bus_im
  set-points sel : BusSelector  OutputSignals=P_set,Q_set
  meas : Outport
  I : Outport  Port=2
  wires:
  set-points/1 -> set-points sel/1
  network/1 -> network sel/1
  set-points sel/1 -> [P_set]  "<P_set>"
  set-points sel/2 -> [Q_set]  "<Q_set>"
  network sel/1 -> [V_re]  "<V_re>"
  network sel/2 -> [V_im]  "<V_im>"
  network sel/3 -> [P_plant]  "<P_plant>"
  network sel/4 -> [Q_plant]  "<Q_plant>"
  network sel/5 -> [V_bus]  "<V_bus>"
  network sel/6 -> [f]  "<f>"
  network sel/7 -> [V_bus_re]  "<V_bus_re>"
  network sel/8 -> [V_bus_im]  "<V_bus_im>"
  [P_set] -> P_set link/1(In1)
  P_set link/1(Out1) -> SPPC/1
  [Q_set] -> Q_set link/1(In1)
  Q_set link/1(Out1) -> SPPC/2
  [P_plant] -> P this plant/1
  P this plant/1 -> P_meas link/1(In1)
  P_meas link/1(Out1) -> SPPC/3
  [Q_plant] -> Q this plant/1
  Q this plant/1 -> Q_meas link/1(In1)
  Q_meas link/1(Out1) -> SPPC/4
  [V_bus] -> V_meas link/1(In1)
  V_meas link/1(Out1) -> SPPC/5
  [P_avail_k] -> P_avail_k link/1(In1)
  P_avail_k link/1(Out1) -> SPPC/6
  [V_bus_re] -> meter/1
  [V_bus_im] -> meter/2
  [f] -> meter/3
  meter/1 -> [f_plant]  "f_plant"
  meter/2 -> RoCoF unused/1  "RoCoF"
  [f_plant] -> f_meas link/1(In1)
  f_meas link/1(Out1) -> SPPC/7
  SPPC/1 -> P_set_k link/1(In1)
  P_set_k link/1(Out1) -> [P_set_k]
  SPPC/2 -> Q_set_k link/1(In1)
  Q_set_k link/1(Out1) -> [Q_set_k]
  [P_set_k] -> P_set_k 1/1
  P_set_k 1/1 -> PV 1/1
  [Q_set_k] -> Q_set_k 1/1
  Q_set_k 1/1 -> PV 1/2
  [V_re] -> V_re 1/1
  V_re 1/1 -> PV 1/3
  [V_im] -> V_im 1/1
  V_im 1/1 -> PV 1/4
  irradiance 1/1 -> PV 1/5
  PV 1/1 -> PV 1 P unused/1
  PV 1/2 -> PV 1 Q unused/1
  PV 1/3 -> [P_avail_1]
  PV 1/4 -> [I_re_1]
  PV 1/5 -> [I_im_1]
  [P_set_k] -> P_set_k 2/1
  P_set_k 2/1 -> PV 2/1
  [Q_set_k] -> Q_set_k 2/1
  Q_set_k 2/1 -> PV 2/2
  [V_re] -> V_re 2/1
  V_re 2/1 -> PV 2/3
  [V_im] -> V_im 2/1
  V_im 2/1 -> PV 2/4
  irradiance 2/1 -> PV 2/5
  PV 2/1 -> PV 2 P unused/1
  PV 2/2 -> PV 2 Q unused/1
  PV 2/3 -> [P_avail_2]
  PV 2/4 -> [I_re_2]
  PV 2/5 -> [I_im_2]
  [P_avail_1] -> P_avail_k/1
  [P_avail_2] -> P_avail_k/2
  [I_re_1] -> I_re_k/1
  [I_re_2] -> I_re_k/2
  [I_im_1] -> I_im_k/1
  [I_im_2] -> I_im_k/2
  P_avail_k/1 -> [P_avail_k]  "P_avail_k"
  I_re_k/1 -> I_re to system pu link/1(In1)  "I_re_k"
  I_im_k/1 -> I_im to system pu link/1(In1)  "I_im_k"
  I_re to system pu link/1(Out1) -> injection/1  "I_re"
  I_im to system pu link/1(Out1) -> injection/2  "I_im"
  injection/1 -> I/1
  SPPC/3 -> P_avail to W link/1(In1)
  P_avail to W link/1(Out1) -> meas bus/1  "P_avail"
  SPPC/4 -> P to W link/1(In1)
  P to W link/1(Out1) -> meas bus/2  "P"
  SPPC/5 -> Q to W link/1(In1)
  Q to W link/1(Out1) -> meas bus/3  "Q"
  SPPC/6 -> meas bus/4  "Q_sat"
  [f_plant] -> meas bus/5  "f_meas"
  meas bus/1 -> meas/1

== system HPP/TSO ==
  f_meas : Inport
  P_ref : Step  Time=p.grid.Pstep.t0  InitialValue=p.grid.Pref  FinalValue=p.grid.Pref + p.grid.Pstep.dP  SampleTime=0
  Q_ref : Step  Time=p.grid.Qstep.t0  InitialValue=p.grid.Qref  FinalValue=p.grid.Qref + p.grid.Qstep.dQ  SampleTime=0
  TSO bus : BusCreator  Inputs=3
  TSO : Outport
  wires:
  P_ref/1 -> TSO bus/1  "P_ref"
  Q_ref/1 -> TSO bus/2  "Q_ref"
  f_meas/1 -> TSO bus/3  "f_meas"
  TSO bus/1 -> TSO/1

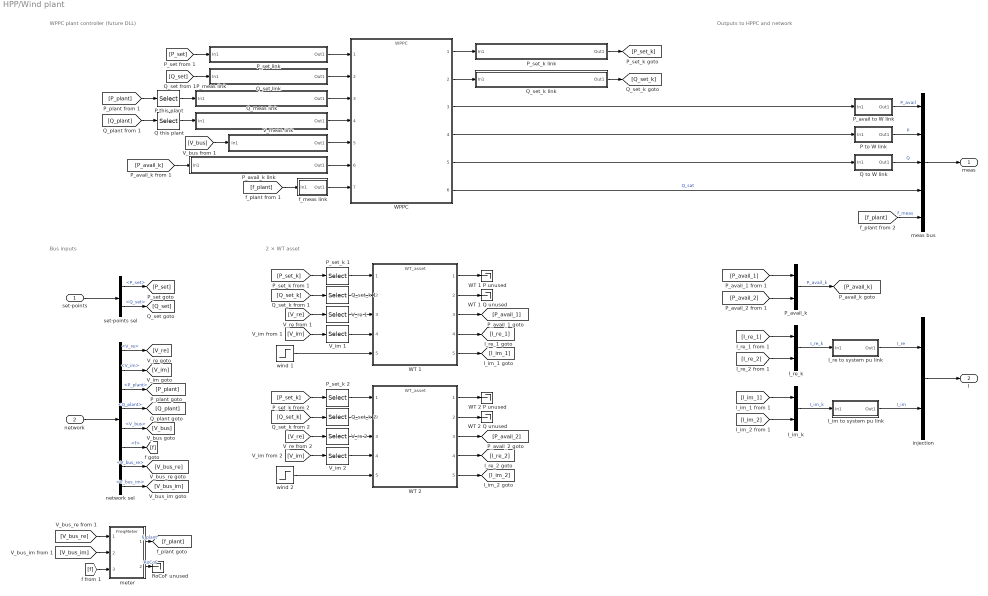
== system HPP/Wind plant ==
  note: Bus inputs
  note: WPPC plant controller (future DLL)
  note: 2 × WT asset
  note: Outputs to HPPC and network
  set-points : Inport
  network : Inport  Port=2
  I_im to system pu link : Subsystem
      mask help: Link: gain p.ctrl.wt.Pbase/p.grid.Pbase.
      mask Display: disp('pu base')
  I_im_k : Mux  Inputs=2
  I_re to system pu link : Subsystem
      mask help: Link: gain p.ctrl.wt.Pbase/p.grid.Pbase.
      mask Display: disp('pu base')
  I_re_k : Mux  Inputs=2
  P this plant : Selector  InputPortWidth=3  IndexOptions=Index vector (dialog)  Indices=1  OutputSizes=1
  P to W link : Subsystem
      mask help: Link: gain p.ctrl.wppc.Pbase.
      mask Display: disp('to SI')
  P_avail to W link : Subsystem
      mask help: Link: gain p.ctrl.wppc.Pbase.
      mask Display: disp('to SI')
  P_avail_k : Mux  Inputs=2
  P_avail_k link : Subsystem
      mask help: Link: gain p.ctrl.wt.Pbase/p.ctrl.wppc.Pbase, then one-step memory, then delay p.comm.meas_plant in whole steps (initial output 0).
      mask Display: disp('pu base | mem | comm.meas_plant')
  P_meas link : Subsystem
      mask help: Link: gain 1/p.ctrl.wppc.Pbase, then one-step memory, then delay p.comm.meas_plant in whole steps (initial output 0).
      mask Display: disp('to pu | mem | comm.meas_plant')
  P_set link : Subsystem
      mask help: Link: delay p.comm.hppc_to_plant in whole steps (initial output 0), then gain 1/p.ctrl.wppc.Pbase.
      mask Display: disp('comm.hppc_to_plant | to pu')
  P_set_k 1 : Selector  InputPortWidth=2  IndexOptions=Index vector (dialog)  Indices=1  OutputSizes=1
  P_set_k 2 : Selector  InputPortWidth=2  IndexOptions=Index vector (dialog)  Indices=2  OutputSizes=1
  P_set_k link : Subsystem
      mask help: Link: delay p.comm.plant_to_asset in whole steps (initial output 0), then gain p.ctrl.wppc.Pbase/p.ctrl.wt.Pbase.
      mask Display: disp('comm.plant_to_asset | pu base')
  Q this plant : Selector  InputPortWidth=3  IndexOptions=Index vector (dialog)  Indices=1  OutputSizes=1
  Q to W link : Subsystem
      mask help: Link: gain p.ctrl.wppc.Pbase.
      mask Display: disp('to SI')
  Q_meas link : Subsystem
      mask help: Link: gain 1/p.ctrl.wppc.Pbase, then one-step memory, then delay p.comm.meas_plant in whole steps (initial output 0).
      mask Display: disp('to pu | mem | comm.meas_plant')
  Q_set link : Subsystem
      mask help: Link: delay p.comm.hppc_to_plant in whole steps (initial output 0), then gain 1/p.ctrl.wppc.Pbase.
      mask Display: disp('comm.hppc_to_plant | to pu')
  Q_set_k 1 : Selector  InputPortWidth=2  IndexOptions=Index vector (dialog)  Indices=1  OutputSizes=1
  Q_set_k 2 : Selector  InputPortWidth=2  IndexOptions=Index vector (dialog)  Indices=2  OutputSizes=1
  Q_set_k link : Subsystem
      mask help: Link: delay p.comm.plant_to_asset in whole steps (initial output 0), then gain p.ctrl.wppc.Pbase/p.ctrl.wt.Pbase.
      mask Display: disp('comm.plant_to_asset | pu base')
  RoCoF unused : Terminator
  V_im 1 : Selector  InputPortWidth=5  IndexOptions=Index vector (dialog)  Indices=1  OutputSizes=1
  V_im 2 : Selector  InputPortWidth=5  IndexOptions=Index vector (dialog)  Indices=2  OutputSizes=1
  V_meas link : Subsystem
      mask help: Link: one-step memory, then delay p.comm.meas_plant in whole steps (initial output 1).
      mask Display: disp('mem | comm.meas_plant')
  V_re 1 : Selector  InputPortWidth=5  IndexOptions=Index vector (dialog)  Indices=1  OutputSizes=1
  V_re 2 : Selector  InputPortWidth=5  IndexOptions=Index vector (dialog)  Indices=2  OutputSizes=1
  WPPC : ModelReference  ModelNameDialog=WPPC  ParameterArgumentNames=par  ParameterArgumentValues=p.ctrl.wppc.par  UsingDefaultArgumentValue=0  SimulationMode=Normal  ModelReferenceVersion=1.1
  WT 1 : ModelReference  ModelNameDialog=WT_asset  ParameterArgumentNames=ap  ParameterArgumentValues=p.wt.ap(1)  UsingDefaultArgumentValue=0  SimulationMode=Normal  ModelReferenceVersion=1.1
  WT 1 P unused : Terminator
  WT 1 Q unused : Terminator
  WT 2 : ModelReference  ModelNameDialog=WT_asset  ParameterArgumentNames=ap  ParameterArgumentValues=p.wt.ap(2)  UsingDefaultArgumentValue=0  SimulationMode=Normal  ModelReferenceVersion=1.1
  WT 2 P unused : Terminator
  WT 2 Q unused : Terminator
  f_meas link : Subsystem
      mask help: Link: one-step memory.
      mask Display: disp('mem')
  injection : BusCreator  Inputs=2
  meas bus : BusCreator  Inputs=5
  meter : ModelReference  ModelNameDialog=FreqMeter  ParameterArgumentNames=m  ParameterArgumentValues=p.pll.wppc  UsingDefaultArgumentValue=0  SimulationMode=Normal  ModelReferenceVersion=1.1
  network sel : BusSelector  OutputSignals=V_re,V_im,P_plant,Q_plant,V_bus,f,V_bus_re,V_bus_im
  set-points sel : BusSelector  OutputSignals=P_set,Q_set
  wind 1 : Step  Time=p.wt.tStep  InitialValue=p.wt.Pavail0  FinalValue=p.wt.PavailStep  SampleTime=0
  wind 2 : Step  Time=p.wt.tStep  InitialValue=p.wt.Pavail0  FinalValue=p.wt.PavailStep  SampleTime=0
  meas : Outport
  I : Outport  Port=2
  wires:
  set-points/1 -> set-points sel/1
  network/1 -> network sel/1
  set-points sel/1 -> [P_set]  "<P_set>"
  set-points sel/2 -> [Q_set]  "<Q_set>"
  network sel/1 -> [V_re]  "<V_re>"
  network sel/2 -> [V_im]  "<V_im>"
  network sel/3 -> [P_plant]  "<P_plant>"
  network sel/4 -> [Q_plant]  "<Q_plant>"
  network sel/5 -> [V_bus]  "<V_bus>"
  network sel/6 -> [f]  "<f>"
  network sel/7 -> [V_bus_re]  "<V_bus_re>"
  network sel/8 -> [V_bus_im]  "<V_bus_im>"
  [P_set] -> P_set link/1(In1)
  P_set link/1(Out1) -> WPPC/1
  [Q_set] -> Q_set link/1(In1)
  Q_set link/1(Out1) -> WPPC/2
  [P_plant] -> P this plant/1
  P this plant/1 -> P_meas link/1(In1)
  P_meas link/1(Out1) -> WPPC/3
  [Q_plant] -> Q this plant/1
  Q this plant/1 -> Q_meas link/1(In1)
  Q_meas link/1(Out1) -> WPPC/4
  [V_bus] -> V_meas link/1(In1)
  V_meas link/1(Out1) -> WPPC/5
  [P_avail_k] -> P_avail_k link/1(In1)
  P_avail_k link/1(Out1) -> WPPC/6
  [V_bus_re] -> meter/1
  [V_bus_im] -> meter/2
  [f] -> meter/3
  meter/1 -> [f_plant]  "f_plant"
  meter/2 -> RoCoF unused/1  "RoCoF"
  [f_plant] -> f_meas link/1(In1)
  f_meas link/1(Out1) -> WPPC/7
  WPPC/1 -> P_set_k link/1(In1)
  P_set_k link/1(Out1) -> [P_set_k]
  WPPC/2 -> Q_set_k link/1(In1)
  Q_set_k link/1(Out1) -> [Q_set_k]
  [P_set_k] -> P_set_k 1/1
  P_set_k 1/1 -> WT 1/1
  [Q_set_k] -> Q_set_k 1/1
  Q_set_k 1/1 -> WT 1/2
  [V_re] -> V_re 1/1
  V_re 1/1 -> WT 1/3
  [V_im] -> V_im 1/1
  V_im 1/1 -> WT 1/4
  wind 1/1 -> WT 1/5
  WT 1/1 -> WT 1 P unused/1
  WT 1/2 -> WT 1 Q unused/1
  WT 1/3 -> [P_avail_1]
  WT 1/4 -> [I_re_1]
  WT 1/5 -> [I_im_1]
  [P_set_k] -> P_set_k 2/1
  P_set_k 2/1 -> WT 2/1
  [Q_set_k] -> Q_set_k 2/1
  Q_set_k 2/1 -> WT 2/2
  [V_re] -> V_re 2/1
  V_re 2/1 -> WT 2/3
  [V_im] -> V_im 2/1
  V_im 2/1 -> WT 2/4
  wind 2/1 -> WT 2/5
  WT 2/1 -> WT 2 P unused/1
  WT 2/2 -> WT 2 Q unused/1
  WT 2/3 -> [P_avail_2]
  WT 2/4 -> [I_re_2]
  WT 2/5 -> [I_im_2]
  [P_avail_1] -> P_avail_k/1
  [P_avail_2] -> P_avail_k/2
  [I_re_1] -> I_re_k/1
  [I_re_2] -> I_re_k/2
  [I_im_1] -> I_im_k/1
  [I_im_2] -> I_im_k/2
  P_avail_k/1 -> [P_avail_k]  "P_avail_k"
  I_re_k/1 -> I_re to system pu link/1(In1)  "I_re_k"
  I_im_k/1 -> I_im to system pu link/1(In1)  "I_im_k"
  I_re to system pu link/1(Out1) -> injection/1  "I_re"
  I_im to system pu link/1(Out1) -> injection/2  "I_im"
  injection/1 -> I/1
  WPPC/3 -> P_avail to W link/1(In1)
  P_avail to W link/1(Out1) -> meas bus/1  "P_avail"
  WPPC/4 -> P to W link/1(In1)
  P to W link/1(Out1) -> meas bus/2  "P"
  WPPC/5 -> Q to W link/1(In1)
  Q to W link/1(Out1) -> meas bus/3  "Q"
  WPPC/6 -> meas bus/4  "Q_sat"
  [f_plant] -> meas bus/5  "f_meas"
  meas bus/1 -> meas/1

== system HPP/BESS plant/I_im to system pu link ==
  In1 : Inport
  gain 1 : Gain  Gain=p.ctrl.bess.Pbase/p.grid.Pbase
  Out1 : Outport
  wires:
  In1/1 -> gain 1/1
  gain 1/1 -> Out1/1

== system HPP/BESS plant/I_re to system pu link ==
  In1 : Inport
  gain 1 : Gain  Gain=p.ctrl.bess.Pbase/p.grid.Pbase
  Out1 : Outport
  wires:
  In1/1 -> gain 1/1
  gain 1/1 -> Out1/1

== system HPP/BESS plant/P to W link ==
  In1 : Inport
  gain 1 : Gain  Gain=p.ctrl.bessc.Pbase
  Out1 : Outport
  wires:
  In1/1 -> gain 1/1
  gain 1/1 -> Out1/1

== system HPP/BESS plant/P_avail_k link ==
  In1 : Inport
  delay 3 : Subsystem  Description=Communication delay of p.comm.steps.meas_plant steps, chosen per run: Fixed (HPP_delays = 1, length fixed at compile time, fastest) or Variable (HPP_delays = 2, tunable up to p.comm.maxDelay). See commParameters, comm.delays.  Variant=on
  gain 1 : Gain  Gain=p.ctrl.bess.Pbase/p.ctrl.bessc.Pbase
  memory 2 : Memory
  Out1 : Outport
  wires:
  In1/1 -> gain 1/1
  delay 3/1(y) -> Out1/1
  memory 2/1 -> delay 3/1(u)
  gain 1/1 -> memory 2/1

== system HPP/BESS plant/P_chg_max to W link ==
  In1 : Inport
  gain 1 : Gain  Gain=p.ctrl.bessc.Pbase
  Out1 : Outport
  wires:
  In1/1 -> gain 1/1
  gain 1/1 -> Out1/1

== system HPP/BESS plant/P_dis_max to W link ==
  In1 : Inport
  gain 1 : Gain  Gain=p.ctrl.bessc.Pbase
  Out1 : Outport
  wires:
  In1/1 -> gain 1/1
  gain 1/1 -> Out1/1

== system HPP/BESS plant/P_meas link ==
  In1 : Inport
  delay 3 : Subsystem  Description=Communication delay of p.comm.steps.meas_plant steps, chosen per run: Fixed (HPP_delays = 1, length fixed at compile time, fastest) or Variable (HPP_delays = 2, tunable up to p.comm.maxDelay). See commParameters, comm.delays.  Variant=on
  gain 1 : Gain  Gain=1/p.ctrl.bessc.Pbase
  memory 2 : Memory
  Out1 : Outport
  wires:
  memory 2/1 -> delay 3/1(u)
  gain 1/1 -> memory 2/1
  In1/1 -> gain 1/1
  delay 3/1(y) -> Out1/1

== system HPP/BESS plant/P_set link ==
  In1 : Inport
  delay 1 : Subsystem  Description=Communication delay of p.comm.steps.hppc_to_plant steps, chosen per run: Fixed (HPP_delays = 1, length fixed at compile time, fastest) or Variable (HPP_delays = 2, tunable up to p.comm.maxDelay). See commParameters, comm.delays.  Variant=on
  gain 2 : Gain  Gain=1/p.ctrl.bessc.Pbase
  Out1 : Outport
  wires:
  delay 1/1(y) -> gain 2/1
  In1/1 -> delay 1/1(u)
  gain 2/1 -> Out1/1

== system HPP/BESS plant/P_set_k link ==
  In1 : Inport
  delay 1 : Subsystem  Description=Communication delay of p.comm.steps.plant_to_asset steps, chosen per run: Fixed (HPP_delays = 1, length fixed at compile time, fastest) or Variable (HPP_delays = 2, tunable up to p.comm.maxDelay). See commParameters, comm.delays.  Variant=on
  gain 2 : Gain  Gain=p.ctrl.bessc.Pbase/p.ctrl.bess.Pbase
  Out1 : Outport
  wires:
  In1/1 -> delay 1/1(u)
  delay 1/1(y) -> gain 2/1
  gain 2/1 -> Out1/1

== system HPP/BESS plant/Q to W link ==
  In1 : Inport
  gain 1 : Gain  Gain=p.ctrl.bessc.Pbase
  Out1 : Outport
  wires:
  In1/1 -> gain 1/1
  gain 1/1 -> Out1/1

== system HPP/BESS plant/Q_meas link ==
  In1 : Inport
  delay 3 : Subsystem  Description=Communication delay of p.comm.steps.meas_plant steps, chosen per run: Fixed (HPP_delays = 1, length fixed at compile time, fastest) or Variable (HPP_delays = 2, tunable up to p.comm.maxDelay). See commParameters, comm.delays.  Variant=on
  gain 1 : Gain  Gain=1/p.ctrl.bessc.Pbase
  memory 2 : Memory
  Out1 : Outport
  wires:
  delay 3/1(y) -> Out1/1
  memory 2/1 -> delay 3/1(u)
  gain 1/1 -> memory 2/1
  In1/1 -> gain 1/1

== system HPP/BESS plant/Q_set link ==
  In1 : Inport
  delay 1 : Subsystem  Description=Communication delay of p.comm.steps.hppc_to_plant steps, chosen per run: Fixed (HPP_delays = 1, length fixed at compile time, fastest) or Variable (HPP_delays = 2, tunable up to p.comm.maxDelay). See commParameters, comm.delays.  Variant=on
  gain 2 : Gain  Gain=1/p.ctrl.bessc.Pbase
  Out1 : Outport
  wires:
  In1/1 -> delay 1/1(u)
  delay 1/1(y) -> gain 2/1
  gain 2/1 -> Out1/1

== system HPP/BESS plant/Q_set_k link ==
  In1 : Inport
  delay 1 : Subsystem  Description=Communication delay of p.comm.steps.plant_to_asset steps, chosen per run: Fixed (HPP_delays = 1, length fixed at compile time, fastest) or Variable (HPP_delays = 2, tunable up to p.comm.maxDelay). See commParameters, comm.delays.  Variant=on
  gain 2 : Gain  Gain=p.ctrl.bessc.Pbase/p.ctrl.bess.Pbase
  Out1 : Outport
  wires:
  In1/1 -> delay 1/1(u)
  delay 1/1(y) -> gain 2/1
  gain 2/1 -> Out1/1

== system HPP/BESS plant/SOC_k link ==
  In1 : Inport
  delay 2 : Subsystem  Description=Communication delay of p.comm.steps.meas_plant steps, chosen per run: Fixed (HPP_delays = 1, length fixed at compile time, fastest) or Variable (HPP_delays = 2, tunable up to p.comm.maxDelay). See commParameters, comm.delays.  Variant=on
  memory 1 : Memory
  Out1 : Outport
  wires:
  In1/1 -> memory 1/1
  delay 2/1(y) -> Out1/1
  memory 1/1 -> delay 2/1(u)

== system HPP/BESS plant/V_meas link ==
  In1 : Inport
  delay 2 : Subsystem  Description=Communication delay of p.comm.steps.meas_plant steps, chosen per run: Fixed (HPP_delays = 1, length fixed at compile time, fastest) or Variable (HPP_delays = 2, tunable up to p.comm.maxDelay). See commParameters, comm.delays.  Variant=on
  memory 1 : Memory
  Out1 : Outport
  wires:
  In1/1 -> memory 1/1
  delay 2/1(y) -> Out1/1
  memory 1/1 -> delay 2/1(u)

== system HPP/BESS plant/f_meas link ==
  In1 : Inport
  memory 1 : Memory
  Out1 : Outport
  wires:
  In1/1 -> memory 1/1
  memory 1/1 -> Out1/1

== system HPP/HPP controller/P_avail_spp link ==
  In1 : Inport
  delay 3 : Subsystem  Description=Communication delay of p.comm.steps.meas_hppc steps, chosen per run: Fixed (HPP_delays = 1, length fixed at compile time, fastest) or Variable (HPP_delays = 2, tunable up to p.comm.maxDelay). See commParameters, comm.delays.  Variant=on
  gain 1 : Gain  Gain=1/p.ctrl.hppc.Pbase
  memory 2 : Memory
  Out1 : Outport
  wires:
  In1/1 -> gain 1/1
  delay 3/1(y) -> Out1/1
  memory 2/1 -> delay 3/1(u)
  gain 1/1 -> memory 2/1

== system HPP/HPP controller/P_avail_wpp link ==
  In1 : Inport
  delay 3 : Subsystem  Description=Communication delay of p.comm.steps.meas_hppc steps, chosen per run: Fixed (HPP_delays = 1, length fixed at compile time, fastest) or Variable (HPP_delays = 2, tunable up to p.comm.maxDelay). See commParameters, comm.delays.  Variant=on
  gain 1 : Gain  Gain=1/p.ctrl.hppc.Pbase
  memory 2 : Memory
  Out1 : Outport
  wires:
  In1/1 -> gain 1/1
  delay 3/1(y) -> Out1/1
  memory 2/1 -> delay 3/1(u)
  gain 1/1 -> memory 2/1

== system HPP/HPP controller/P_bess link ==
  In1 : Inport
  delay 3 : Subsystem  Description=Communication delay of p.comm.steps.meas_hppc steps, chosen per run: Fixed (HPP_delays = 1, length fixed at compile time, fastest) or Variable (HPP_delays = 2, tunable up to p.comm.maxDelay). See commParameters, comm.delays.  Variant=on
  gain 1 : Gain  Gain=1/p.ctrl.hppc.Pbase
  memory 2 : Memory
  Out1 : Outport
  wires:
  In1/1 -> gain 1/1
  delay 3/1(y) -> Out1/1
  memory 2/1 -> delay 3/1(u)
  gain 1/1 -> memory 2/1

== system HPP/HPP controller/P_chg_max_bess link ==
  In1 : Inport
  delay 3 : Subsystem  Description=Communication delay of p.comm.steps.meas_hppc steps, chosen per run: Fixed (HPP_delays = 1, length fixed at compile time, fastest) or Variable (HPP_delays = 2, tunable up to p.comm.maxDelay). See commParameters, comm.delays.  Variant=on
  gain 1 : Gain  Gain=1/p.ctrl.hppc.Pbase
  memory 2 : Memory
  Out1 : Outport
  wires:
  In1/1 -> gain 1/1
  delay 3/1(y) -> Out1/1
  memory 2/1 -> delay 3/1(u)
  gain 1/1 -> memory 2/1

== system HPP/HPP controller/P_dis_max_bess link ==
  In1 : Inport
  delay 3 : Subsystem  Description=Communication delay of p.comm.steps.meas_hppc steps, chosen per run: Fixed (HPP_delays = 1, length fixed at compile time, fastest) or Variable (HPP_delays = 2, tunable up to p.comm.maxDelay). See commParameters, comm.delays.  Variant=on
  gain 1 : Gain  Gain=1/p.ctrl.hppc.Pbase
  memory 2 : Memory
  Out1 : Outport
  wires:
  In1/1 -> gain 1/1
  delay 3/1(y) -> Out1/1
  memory 2/1 -> delay 3/1(u)
  gain 1/1 -> memory 2/1

== system HPP/HPP controller/P_poc link ==
  In1 : Inport
  delay 3 : Subsystem  Description=Communication delay of p.comm.steps.meas_hppc steps, chosen per run: Fixed (HPP_delays = 1, length fixed at compile time, fastest) or Variable (HPP_delays = 2, tunable up to p.comm.maxDelay). See commParameters, comm.delays.  Variant=on
  gain 1 : Gain  Gain=1/p.ctrl.hppc.Pbase
  memory 2 : Memory
  Out1 : Outport
  wires:
  In1/1 -> gain 1/1
  gain 1/1 -> memory 2/1
  delay 3/1(y) -> Out1/1
  memory 2/1 -> delay 3/1(u)

== system HPP/HPP controller/P_ref link ==
  In1 : Inport
  delay 2 : Subsystem  Description=Communication delay of p.comm.steps.tso steps, chosen per run: Fixed (HPP_delays = 1, length fixed at compile time, fastest) or Variable (HPP_delays = 2, tunable up to p.comm.maxDelay). See commParameters, comm.delays.  Variant=on
  gain 1 : Gain  Gain=1/p.ctrl.hppc.Pbase
  Out1 : Outport
  wires:
  In1/1 -> gain 1/1
  gain 1/1 -> delay 2/1(u)
  delay 2/1(y) -> Out1/1
